simulink model "crs_controller"  (R2026b)
settings: Solver=FixedStepDiscrete  FixedStep=Ts
undefined symbols (not defined in the file): brake_threshold, DiscIntNeverNeededParam, KeyON, Kp, opMode, reqMode, ShiftDrive, target_dec_hold, target_dec_short, target_inc_hold, target_inc_short, throt_max, throt_min, Ts, tsp_max, tsp_min
libraries: simulink x73
settings Model: DataDictionary=crs_controllerdic.sldd  Creator=The MathWorks, Inc.  LastModifiedBy=alexkim
settings DataIOCC: DSMLogging=off  ReturnWorkspaceOutputs=off  SaveOutput=off  SaveTime=off  SignalLogging=off
settings OptimizationCC: DefaultParameterBehavior=Inlined  EfficientTunableParamExpr=on  PassReuseOutputArgsAs=Individual arguments
settings DebuggingCC: ArithmeticOperatorsInVariantConditions=warning  ParameterTunabilityLossMsg=error
settings SFSimCC: CustomCodeUndefinedFunction=UseInterfaceOnly  SimUseLocalCustomCode=off
settings RTWCC: DLArmComputeVersion=19.05  Description=Embedded Coder  GenCodeOnly=on  GenerateReport=on  GenerateTraceInfo=on  GenerateTraceReport=on  GenerateTraceReportEml=on  GenerateTraceReportSf=on  GenerateTraceReportSl=on  IncludeHyperlinkInReport=on  LaunchReport=on  RTWUseLocalCustomCode=off  SystemTargetFile=ert.tlc  TemplateMakefile=ert_default_tmf
settings CodeAppCC: ForceParamTrailComments=on  IgnoreCustomStorageClasses=off  InsertBlockDesc=on  MATLABFcnDesc=on  MATLABSourceComments=on  OperatorAnnotations=on  ReqsInCode=on  SFDataObjDesc=on  SimulinkDataObjDesc=on  StateflowObjectComments=on
settings ERTTargetCC: DynamicArrayContainerType=coder::array  GenerateSampleERTMain=on

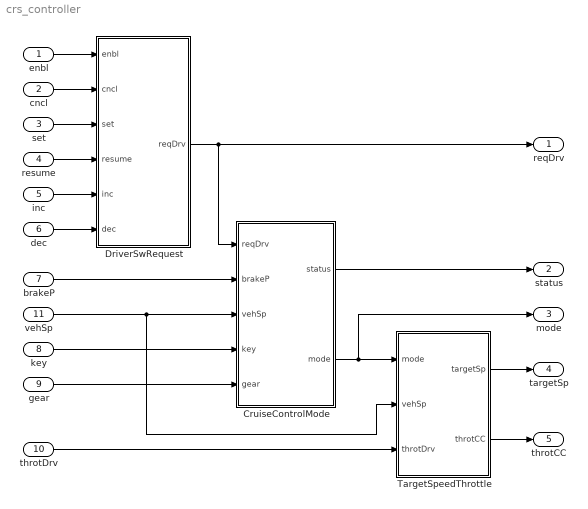
== system crs_controller ==
  enbl : Inport  OutDataTypeStr=boolean
  cncl : Inport  Port=2  OutDataTypeStr=boolean
  set : Inport  Port=3  OutDataTypeStr=boolean
  resume : Inport  Port=4  OutDataTypeStr=boolean
  inc : Inport  Port=5  OutDataTypeStr=boolean
  dec : Inport  Port=6  OutDataTypeStr=boolean
  brakeP : Inport  Port=7
  key : Inport  Port=8
  gear : Inport  Port=9  Interpolate=off
  throtDrv : Inport  Port=10
  vehSp : Inport  Port=11
  CruiseControlMode : Subsystem  RequirementInfo="{}  %GIDa_bb6d1dc8_bb76_4df1_9873_999afa682800"  TreatAsAtomicUnit=on
  DriverSwRequest : Subsystem  RequirementInfo="{}  %GIDa_29e5572c_7fa7_4cd7_a964_a3217c292b35"  TreatAsAtomicUnit=on
  TargetSpeedThrottle : Subsystem  RequirementInfo="{}  %GIDa_aedc9787_ada3_4e37_9146_515463f4d0c7"  TreatAsAtomicUnit=on
  reqDrv : Outport  VectorParamsAs1DForOutWhenUnconnected=off
  status : Outport  Port=2  VectorParamsAs1DForOutWhenUnconnected=off
  mode : Outport  Port=3  VectorParamsAs1DForOutWhenUnconnected=off
  targetSp : Outport  Port=4  VectorParamsAs1DForOutWhenUnconnected=off
  throtCC : Outport  Port=5  VectorParamsAs1DForOutWhenUnconnected=off
  wires:
  dec/1 -> DriverSwRequest/6(dec)
  inc/1 -> DriverSwRequest/5(inc)
  enbl/1 -> DriverSwRequest/1(enbl)
  vehSp/1 -> TargetSpeedThrottle/2(vehSp), CruiseControlMode/3(vehSp)
  CruiseControlMode/2(mode) -> mode/1, TargetSpeedThrottle/1(mode)
  throtDrv/1 -> TargetSpeedThrottle/3(throtDrv)
  TargetSpeedThrottle/2(throtCC) -> throtCC/1
  DriverSwRequest/1(reqDrv) -> reqDrv/1, CruiseControlMode/1(reqDrv)
  resume/1 -> DriverSwRequest/4(resume)
  set/1 -> DriverSwRequest/3(set)
  CruiseControlMode/1(status) -> status/1
  TargetSpeedThrottle/1(targetSp) -> targetSp/1
  gear/1 -> CruiseControlMode/5(gear)
  cncl/1 -> DriverSwRequest/2(cncl)
  brakeP/1 -> CruiseControlMode/2(brakeP)
  key/1 -> CruiseControlMode/4(key)

== system crs_controller/CruiseControlMode ==
  reqDrv : Inport
  brakeP : Inport  Port=2
  vehSp : Inport  Port=3
  key : Inport  Port=4
  gear : Inport  Port=5
  EnumConst2 : simulink/Sources/Enumerated Constant  OutDataTypeStr=Enum: opMode  Value=opMode.Disable  SampleTime=inf
  Switch : Switch  Criteria=u2 ~= 0  SaturateOnIntegerOverflow=off  InputSameDT=off
  UnitDelay : UnitDelay  InitialCondition=opMode.Disable  SampleTime=-1
      settings: AttributesFormatString=Init = %<InitialCondition>
  disableCaseDetection : Subsystem
  getActStatus : Subsystem
  opMode : Subsystem  TreatAsAtomicUnit=on
  outOfRange : Subsystem
  status : Outport  VectorParamsAs1DForOutWhenUnconnected=off
  mode : Outport  Port=2  VectorParamsAs1DForOutWhenUnconnected=off
  wires:
  EnumConst2/1 -> Switch/1
  brakeP/1 -> disableCaseDetection/3(brakeP)
  key/1 -> disableCaseDetection/1(key)
  gear/1 -> disableCaseDetection/2(gear)
  disableCaseDetection/1(disable_flag) -> Switch/2
  reqDrv/1 -> opMode/1(reqDrv)
  UnitDelay/1 -> opMode/3(mode_prev)  "mode_prev"
  getActStatus/1(cc_act_status) -> status/1
  opMode/1(mode) -> Switch/3  "act_mode"
  Switch/1 -> mode/1, getActStatus/1(mode), UnitDelay/1  "mode"
  vehSp/1 -> outOfRange/1(vehSp)
  outOfRange/1(outRange) -> opMode/2(outRange)

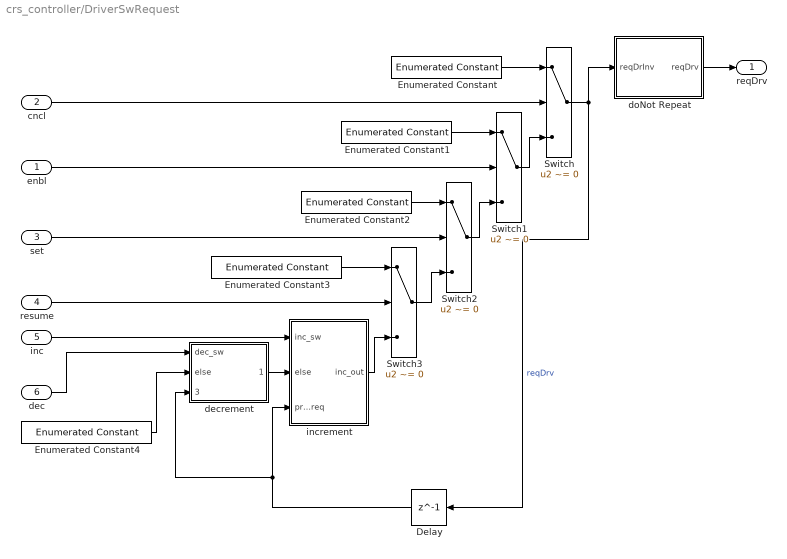
== system crs_controller/DriverSwRequest ==
  enbl : Inport
  cncl : Inport  Port=2
  set : Inport  Port=3
  resume : Inport  Port=4
  inc : Inport  Port=5  OutDataTypeStr=boolean
  dec : Inport  Port=6  OutDataTypeStr=boolean
  Delay : Delay  DelayLength=1  InitialCondition=reqMode.NoRequest
      settings: AttributesFormatString=IC: %<InitialCondition>
  Enumerated Constant : simulink/Sources/Enumerated Constant  OutDataTypeStr=Enum: reqMode  Value=reqMode.Cancel  SampleTime=inf
  Enumerated Constant1 : simulink/Sources/Enumerated Constant  OutDataTypeStr=Enum: reqMode  Value=reqMode.Cruise  SampleTime=inf
  Enumerated Constant2 : simulink/Sources/Enumerated Constant  OutDataTypeStr=Enum: reqMode  Value=reqMode.Set  SampleTime=inf
  Enumerated Constant3 : simulink/Sources/Enumerated Constant  OutDataTypeStr=Enum: reqMode  Value=reqMode.ResumeReq  SampleTime=inf
  Enumerated Constant4 : simulink/Sources/Enumerated Constant  OutDataTypeStr=Enum: reqMode  Value=reqMode.NoRequest  SampleTime=inf
  Switch : Switch  RequirementInfo="{}  %GIDa_5d0d916b_47a2_4532_93c1_fba9212dd833"  Criteria=u2 ~= 0  SaturateOnIntegerOverflow=off  InputSameDT=off
  Switch1 : Switch  RequirementInfo="{}  %GIDa_9aa713f9_64ac_4216_9525_3a0940fa8516"  Criteria=u2 ~= 0  SaturateOnIntegerOverflow=off  InputSameDT=off
  Switch2 : Switch  Criteria=u2 ~= 0  SaturateOnIntegerOverflow=off  InputSameDT=off
  Switch3 : Switch  Criteria=u2 ~= 0  SaturateOnIntegerOverflow=off  InputSameDT=off
  decrement : Subsystem
  doNot Repeat : Subsystem
  increment : Subsystem
  reqDrv : Outport  VectorParamsAs1DForOutWhenUnconnected=off
  wires:
  Enumerated Constant/1 -> Switch/1
  Switch/1 -> doNot Repeat/1(reqDrInv), Delay/1  "reqDrv"
  cncl/1 -> Switch/2
  enbl/1 -> Switch1/2
  Enumerated Constant1/1 -> Switch1/1
  Switch1/1 -> Switch/3
  set/1 -> Switch2/2
  Enumerated Constant2/1 -> Switch2/1
  resume/1 -> Switch3/2
  Enumerated Constant3/1 -> Switch3/1
  Switch3/1 -> Switch2/3
  Switch2/1 -> Switch1/3
  dec/1 -> decrement/1(dec_sw)
  Enumerated Constant4/1 -> decrement/2(else)
  inc/1 -> increment/1(inc_sw)
  decrement/1(dec_out) -> increment/2(else)
  increment/1(inc_out) -> Switch3/3
  Delay/1 -> increment/3(prev_req), decrement/3(prev_req)
  doNot Repeat/1(reqDrv) -> reqDrv/1

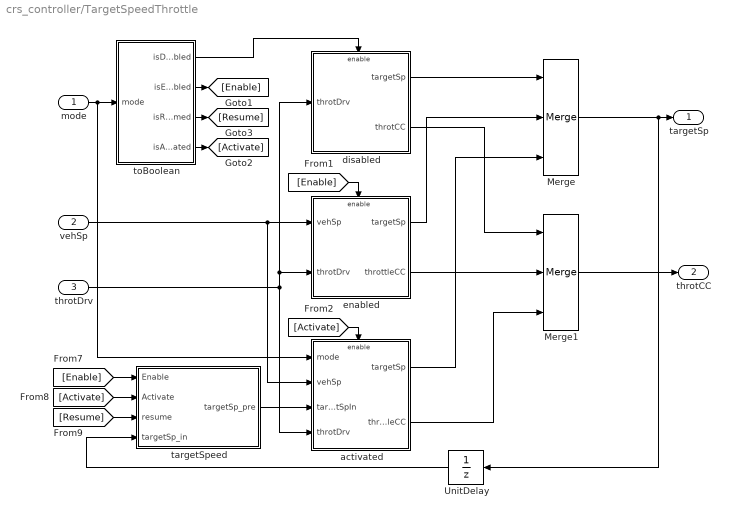
== system crs_controller/TargetSpeedThrottle ==
  mode : Inport
  vehSp : Inport  Port=2
  throtDrv : Inport  Port=3
  Merge : Merge  Inputs=3
  Merge1 : Merge  Inputs=3
  UnitDelay : UnitDelay  SampleTime=-1
      settings: AttributesFormatString=Init = %<InitialCondition>
  activated : Subsystem  TreatAsAtomicUnit=on
  disabled : Subsystem  TreatAsAtomicUnit=on
  enabled : Subsystem  TreatAsAtomicUnit=on
  targetSpeed : Subsystem
  toBoolean : Subsystem
  targetSp : Outport  VectorParamsAs1DForOutWhenUnconnected=off
  throtCC : Outport  Port=2  VectorParamsAs1DForOutWhenUnconnected=off
  wires:
  [Activate] -> targetSpeed/2(Activate)
  [Enable] -> targetSpeed/1(Enable)
  targetSpeed/1(targetSp_pre) -> activated/3(targetSpIn)
  mode/1 -> toBoolean/1(mode), activated/1(mode)
  [Activate] -> activated/Enable
  [Enable] -> enabled/Enable
  toBoolean/1(isDisabled) -> disabled/Enable
  UnitDelay/1 -> targetSpeed/4(targetSp_in)
  Merge/1 -> targetSp/1, UnitDelay/1
  throtDrv/1 -> disabled/1(throtDrv), enabled/2(throtDrv), activated/4(throtDrv)
  vehSp/1 -> activated/2(vehSp), enabled/1(vehSp)
  toBoolean/2(isEnabled) -> [Enable]
  toBoolean/3(isResumed) -> [Resume]
  toBoolean/4(isActivated) -> [Activate]
  [Resume] -> targetSpeed/3(resume)
  disabled/1(targetSp) -> Merge/1
  enabled/1(targetSp) -> Merge/2
  activated/1(targetSp) -> Merge/3
  activated/2(throttleCC) -> Merge1/3
  enabled/2(throttleCC) -> Merge1/2
  disabled/2(throtCC) -> Merge1/1
  Merge1/1 -> throtCC/1

== system crs_controller/CruiseControlMode/disableCaseDetection ==
  key : Inport
  gear : Inport  Port=2
  brakeP : Inport  Port=3
  IsKeyPositionOn : Subsystem
  IsShiftDrive : Subsystem
  LogicOp1 : Logic  Operator=OR  Inputs=3  AllPortsSameDT=off  OutDataTypeStr=boolean
  isbrake : Subsystem
  disable_flag : Outport  VectorParamsAs1DForOutWhenUnconnected=off
  wires:
  LogicOp1/1 -> disable_flag/1
  brakeP/1 -> isbrake/1(brakeP)
  isbrake/1(isbrake) -> LogicOp1/3  "isbrake"
  key/1 -> IsKeyPositionOn/1(In1)
  IsKeyPositionOn/1(Out1) -> LogicOp1/1
  gear/1 -> IsShiftDrive/1(In1)
  IsShiftDrive/1(Out1) -> LogicOp1/2

== system crs_controller/CruiseControlMode/getActStatus ==
  mode : Inport
  EnumConst1 : simulink/Sources/Enumerated Constant  OutDataTypeStr=Enum: opMode  Value=opMode.Disable  SampleTime=inf
  EnumConst2 : simulink/Sources/Enumerated Constant  OutDataTypeStr=Enum: opMode  Value=opMode.Enable  SampleTime=inf
  LogicOp1 : Logic  AllPortsSameDT=off  OutDataTypeStr=boolean
  Relational Operator1 : RelationalOperator  Operator=~=  OutDataTypeStr=boolean  InputSameDT=off
  Relational Operator2 : RelationalOperator  Operator=~=  OutDataTypeStr=boolean  InputSameDT=off
  cc_act_status : Outport  VectorParamsAs1DForOutWhenUnconnected=off
  wires:
  Relational Operator2/1 -> LogicOp1/1
  EnumConst1/1 -> Relational Operator2/1
  mode/1 -> Relational Operator1/2, Relational Operator2/2
  Relational Operator1/1 -> LogicOp1/2
  EnumConst2/1 -> Relational Operator1/1
  LogicOp1/1 -> cc_act_status/1

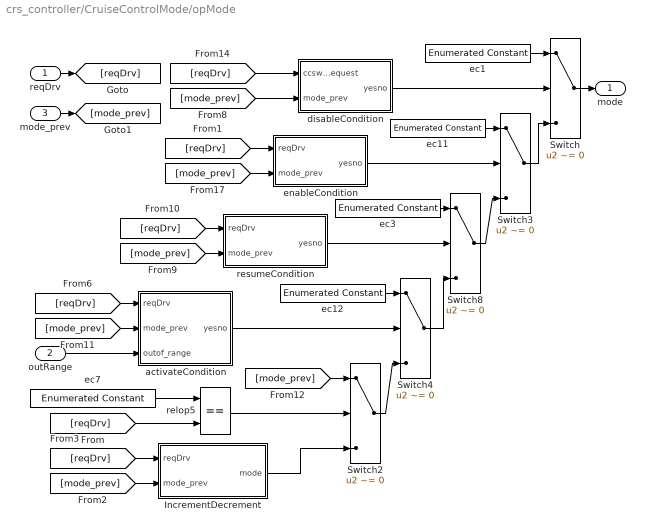
== system crs_controller/CruiseControlMode/opMode ==
  reqDrv : Inport
  outRange : Inport  Port=2
  mode_prev : Inport  Port=3
  IncrementDecrement : Subsystem
  Switch{,2..4,8} (5 alike) : Switch  Criteria=u2 ~= 0  SaturateOnIntegerOverflow=off  InputSameDT=off
  activateCondition : Subsystem
  disableCondition : Subsystem
  ec1 : simulink/Sources/Enumerated Constant  OutDataTypeStr=Enum: opMode  Value=opMode.Disable  SampleTime=inf
  ec11 : simulink/Sources/Enumerated Constant  OutDataTypeStr=Enum: opMode  Value=opMode.Enable  SampleTime=inf
  ec12 : simulink/Sources/Enumerated Constant  OutDataTypeStr=Enum: opMode  Value=opMode.Activate  SampleTime=inf
  ec3 : simulink/Sources/Enumerated Constant  OutDataTypeStr=Enum: opMode  Value=opMode.Resume  SampleTime=inf
  ec7 : simulink/Sources/Enumerated Constant  OutDataTypeStr=Enum: reqMode  Value=reqMode.NoRequest  SampleTime=inf
  enableCondition : Subsystem
  relop5 : RelationalOperator  Operator===  OutDataTypeStr=boolean  InputSameDT=off
  resumeCondition : Subsystem
  mode : Outport  VectorParamsAs1DForOutWhenUnconnected=off
  wires:
  Switch/1 -> mode/1
  ec1/1 -> Switch/1
  ec7/1 -> relop5/1
  ec11/1 -> Switch3/1
  ec12/1 -> Switch4/1
  [reqDrv] -> relop5/2
  [mode_prev] -> Switch2/1
  [reqDrv] -> enableCondition/1(reqDrv)
  mode_prev/1 -> [mode_prev]
  enableCondition/1(yesno) -> Switch3/2
  disableCondition/1(yesno) -> Switch/2
  Switch3/1 -> Switch/3
  activateCondition/1(yesno) -> Switch4/2
  [reqDrv] -> activateCondition/1(reqDrv)
  [mode_prev] -> activateCondition/2(mode_prev)
  [mode_prev] -> disableCondition/2(mode_prev)
  reqDrv/1 -> [reqDrv]
  relop5/1 -> Switch2/2
  Switch2/1 -> Switch4/3
  Switch8/1 -> Switch3/3
  Switch4/1 -> Switch8/3
  resumeCondition/1(yesno) -> Switch8/2
  [mode_prev] -> resumeCondition/2(mode_prev)
  [reqDrv] -> resumeCondition/1(reqDrv)
  ec3/1 -> Switch8/1
  [reqDrv] -> disableCondition/1(ccsw_request)
  outRange/1 -> activateCondition/3(outof_range)
  [mode_prev] -> enableCondition/2(mode_prev)
  [reqDrv] -> IncrementDecrement/1(reqDrv)
  [mode_prev] -> IncrementDecrement/2(mode_prev)
  IncrementDecrement/1(mode) -> Switch2/3

== system crs_controller/CruiseControlMode/outOfRange ==
  vehSp : Inport
  Compare To Constant : simulink/Logic and Bit Operations/Compare To Constant  relop=<  const=tsp_min  OutDataTypeStr=boolean
  Compare To Constant1 : simulink/Logic and Bit Operations/Compare To Constant  relop=>  const=tsp_max  OutDataTypeStr=boolean
  LogicOp : Logic  Operator=OR  AllPortsSameDT=off  OutDataTypeStr=boolean
  outRange : Outport  VectorParamsAs1DForOutWhenUnconnected=off
  wires:
  LogicOp/1 -> outRange/1
  Compare To Constant1/1 -> LogicOp/2
  Compare To Constant/1 -> LogicOp/1
  vehSp/1 -> Compare To Constant/1, Compare To Constant1/1

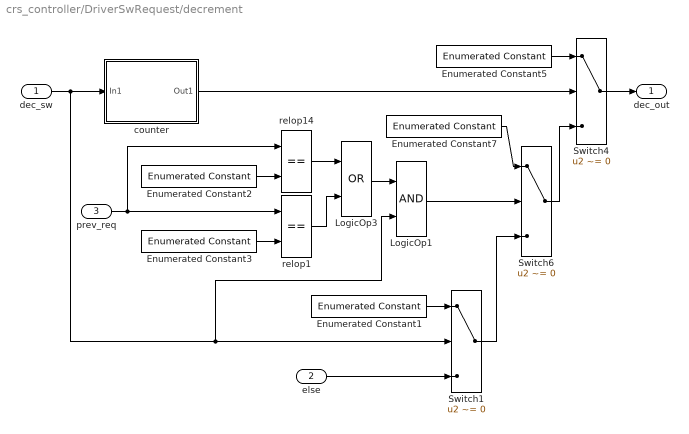
== system crs_controller/DriverSwRequest/decrement ==
  dec_sw : Inport
  else : Inport  Port=2
  prev_req : Inport  Port=3
  Enumerated Constant1 : simulink/Sources/Enumerated Constant  OutDataTypeStr=Enum: reqMode  Value=reqMode.Dec_Short  SampleTime=inf
  Enumerated Constant2 : simulink/Sources/Enumerated Constant  OutDataTypeStr=Enum: reqMode  Value=reqMode.Dec_Short  SampleTime=inf
  Enumerated Constant3 : simulink/Sources/Enumerated Constant  OutDataTypeStr=Enum: reqMode  Value=reqMode.Dec_Middle  SampleTime=inf
  Enumerated Constant5 : simulink/Sources/Enumerated Constant  OutDataTypeStr=Enum: reqMode  Value=reqMode.Dec_Long  SampleTime=inf
  Enumerated Constant7 : simulink/Sources/Enumerated Constant  OutDataTypeStr=Enum: reqMode  Value=reqMode.Dec_Middle  SampleTime=inf
  LogicOp1 : Logic  AllPortsSameDT=off  OutDataTypeStr=boolean
  LogicOp3 : Logic  Operator=OR  AllPortsSameDT=off  OutDataTypeStr=boolean
  Switch1 : Switch  Criteria=u2 ~= 0  SaturateOnIntegerOverflow=off  InputSameDT=off
  Switch4 : Switch  Criteria=u2 ~= 0  SaturateOnIntegerOverflow=off  InputSameDT=off
  Switch6 : Switch  Criteria=u2 ~= 0  SaturateOnIntegerOverflow=off  InputSameDT=off
  counter : Subsystem  DisableCoverage=on  mask(SLDV counter){CountValue=50, OutDataTypeStr=uint8}
      mask prompts: CountValue "Count value"; OutDataTypeStr "Data type"
      mask help: A counter block optimized for Simulink Design Verifier test case generation. If the input is true for consecutive steps which is specified the Count value parameter, then the output is TRUE, otherwise it is FALSE.
      mask init:
      | if CountValue < 0 || CountValue > intmax(OutDataTypeStr)
      |     error('Specified count value needs to be within 0-%d.',intmax(OutDataTypeStr))
      | end
      mask Display: disp(sprintf('Counter (%s)\nCount:%d',OutDataTypeStr,CountValue))
  relop1 : RelationalOperator  Operator===  OutDataTypeStr=boolean  InputSameDT=off
  relop14 : RelationalOperator  Operator===  OutDataTypeStr=boolean  InputSameDT=off
  dec_out : Outport  VectorParamsAs1DForOutWhenUnconnected=off
  wires:
  Enumerated Constant5/1 -> Switch4/1
  Switch4/1 -> dec_out/1
  Enumerated Constant7/1 -> Switch6/1
  Switch6/1 -> Switch4/3
  counter/1(Out1) -> Switch4/2
  Switch1/1 -> Switch6/3
  dec_sw/1 -> counter/1(In1), LogicOp1/2, Switch1/2
  else/1 -> Switch1/3
  Enumerated Constant1/1 -> Switch1/1
  Enumerated Constant2/1 -> relop14/2
  Enumerated Constant3/1 -> relop1/2
  prev_req/1 -> relop14/1, relop1/1
  relop14/1 -> LogicOp3/1
  relop1/1 -> LogicOp3/2
  LogicOp3/1 -> LogicOp1/1
  LogicOp1/1 -> Switch6/2

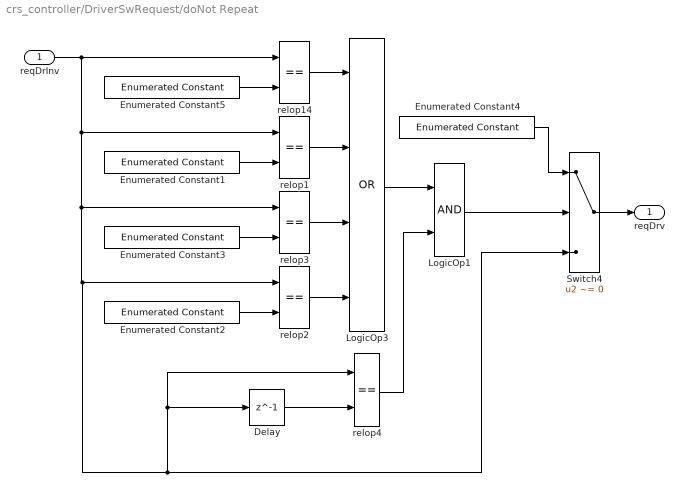
== system crs_controller/DriverSwRequest/doNot Repeat ==
  reqDrInv : Inport
  Delay : Delay  DelayLength=1  InitialCondition=reqMode.NoRequest
      settings: AttributesFormatString=Init = %<InitialCondition>
  Enumerated Constant1 : simulink/Sources/Enumerated Constant  OutDataTypeStr=Enum: reqMode  Value=reqMode.Cruise  SampleTime=inf
  Enumerated Constant2 : simulink/Sources/Enumerated Constant  OutDataTypeStr=Enum: reqMode  Value=reqMode.ResumeReq  SampleTime=inf
  Enumerated Constant3 : simulink/Sources/Enumerated Constant  OutDataTypeStr=Enum: reqMode  Value=reqMode.Set  SampleTime=inf
  Enumerated Constant4 : simulink/Sources/Enumerated Constant  OutDataTypeStr=Enum: reqMode  Value=reqMode.NoRequest  SampleTime=inf
  Enumerated Constant5 : simulink/Sources/Enumerated Constant  OutDataTypeStr=Enum: reqMode  Value=reqMode.Cancel  SampleTime=inf
  LogicOp1 : Logic  AllPortsSameDT=off  OutDataTypeStr=boolean
  LogicOp3 : Logic  Operator=OR  Inputs=4  AllPortsSameDT=off  OutDataTypeStr=boolean
  Switch4 : Switch  Criteria=u2 ~= 0  SaturateOnIntegerOverflow=off  InputSameDT=off
  relop{1..4,14} (5 alike) : RelationalOperator  Operator===  OutDataTypeStr=boolean  InputSameDT=off
  reqDrv : Outport  VectorParamsAs1DForOutWhenUnconnected=off
  wires:
  Enumerated Constant5/1 -> relop14/2
  Enumerated Constant1/1 -> relop1/2
  Enumerated Constant3/1 -> relop3/2
  Enumerated Constant2/1 -> relop2/2
  reqDrInv/1 -> Switch4/3, relop4/1, Delay/1, relop2/1, relop3/1, relop1/1, relop14/1
  relop14/1 -> LogicOp3/1
  relop1/1 -> LogicOp3/2
  relop3/1 -> LogicOp3/3
  relop2/1 -> LogicOp3/4
  Switch4/1 -> reqDrv/1
  Delay/1 -> relop4/2
  relop4/1 -> LogicOp1/2
  LogicOp3/1 -> LogicOp1/1
  LogicOp1/1 -> Switch4/2
  Enumerated Constant4/1 -> Switch4/1

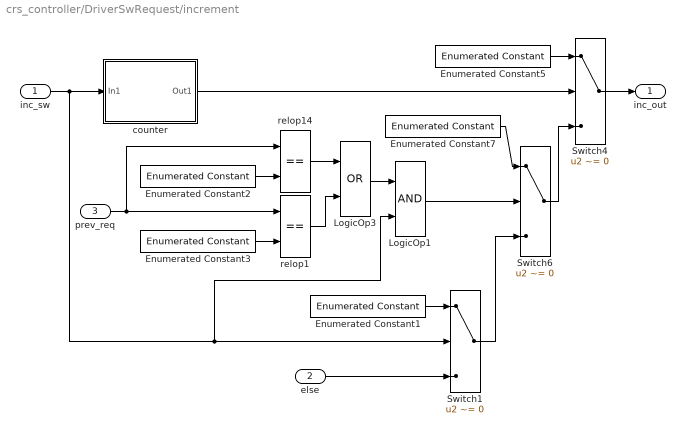
== system crs_controller/DriverSwRequest/increment ==
  inc_sw : Inport
  else : Inport  Port=2
  prev_req : Inport  Port=3
  Enumerated Constant1 : simulink/Sources/Enumerated Constant  OutDataTypeStr=Enum: reqMode  Value=reqMode.Inc_Short  SampleTime=inf
  Enumerated Constant2 : simulink/Sources/Enumerated Constant  OutDataTypeStr=Enum: reqMode  Value=reqMode.Inc_Short  SampleTime=inf
  Enumerated Constant3 : simulink/Sources/Enumerated Constant  OutDataTypeStr=Enum: reqMode  Value=reqMode.Inc_Middle  SampleTime=inf
  Enumerated Constant5 : simulink/Sources/Enumerated Constant  OutDataTypeStr=Enum: reqMode  Value=reqMode.Inc_Long  SampleTime=inf
  Enumerated Constant7 : simulink/Sources/Enumerated Constant  OutDataTypeStr=Enum: reqMode  Value=reqMode.Inc_Middle  SampleTime=inf
  LogicOp1 : Logic  AllPortsSameDT=off  OutDataTypeStr=boolean
  LogicOp3 : Logic  Operator=OR  AllPortsSameDT=off  OutDataTypeStr=boolean
  Switch1 : Switch  Criteria=u2 ~= 0  SaturateOnIntegerOverflow=off  InputSameDT=off
  Switch4 : Switch  Criteria=u2 ~= 0  SaturateOnIntegerOverflow=off  InputSameDT=off
  Switch6 : Switch  Criteria=u2 ~= 0  SaturateOnIntegerOverflow=off  InputSameDT=off
  counter : Subsystem  DisableCoverage=on  mask(SLDV counter){CountValue=50, OutDataTypeStr=uint8}
      mask prompts: CountValue "Count value"; OutDataTypeStr "Data type"
      mask help: A counter block optimized for Simulink Design Verifier test case generation. If the input is true for consecutive steps which is specified the Count value parameter, then the output is TRUE, otherwise it is FALSE.
      mask init:
      | if CountValue < 0 || CountValue > intmax(OutDataTypeStr)
      |     error('Specified count value needs to be within 0-%d.',intmax(OutDataTypeStr))
      | end
      mask Display: disp(sprintf('Counter (%s)\nCount:%d',OutDataTypeStr,CountValue))
  relop1 : RelationalOperator  Operator===  OutDataTypeStr=boolean  InputSameDT=off
  relop14 : RelationalOperator  Operator===  OutDataTypeStr=boolean  InputSameDT=off
  inc_out : Outport  VectorParamsAs1DForOutWhenUnconnected=off
  wires:
  Enumerated Constant5/1 -> Switch4/1
  Switch4/1 -> inc_out/1
  Enumerated Constant7/1 -> Switch6/1
  Switch6/1 -> Switch4/3
  counter/1(Out1) -> Switch4/2
  Switch1/1 -> Switch6/3
  inc_sw/1 -> counter/1(In1), LogicOp1/2, Switch1/2
  else/1 -> Switch1/3
  Enumerated Constant1/1 -> Switch1/1
  Enumerated Constant2/1 -> relop14/2
  Enumerated Constant3/1 -> relop1/2
  prev_req/1 -> relop14/1, relop1/1
  relop14/1 -> LogicOp3/1
  relop1/1 -> LogicOp3/2
  LogicOp3/1 -> LogicOp1/1
  LogicOp1/1 -> Switch6/2

== system crs_controller/TargetSpeedThrottle/activated ==
  mode : Inport
  vehSp : Inport  Port=2
  targetSpIn : Inport  Port=3
  throtDrv : Inport  Port=4
  Enable : EnablePort
  getNewTargetSpeed : Subsystem
  getThrottleValue : Subsystem
  targetSp : Outport  VectorParamsAs1DForOutWhenUnconnected=off
  throttleCC : Outport  Port=2  VectorParamsAs1DForOutWhenUnconnected=off
  wires:
  targetSpIn/1 -> getThrottleValue/1(In1), getNewTargetSpeed/1(targetSpIn)
  mode/1 -> getNewTargetSpeed/2(mode)
  getNewTargetSpeed/1(targetSp) -> targetSp/1  "targetSp"
  vehSp/1 -> getThrottleValue/2(In2)
  throtDrv/1 -> getThrottleValue/3(In3)
  getThrottleValue/1(Out1) -> throttleCC/1

== system crs_controller/TargetSpeedThrottle/disabled ==
  throtDrv : Inport
  Enable : EnablePort
  Constant : Constant  Value=tsp_min  OutDataTypeStr=Inherit: Inherit via back propagation
  targetSp : Outport  VectorParamsAs1DForOutWhenUnconnected=off
  throtCC : Outport  Port=2  VectorParamsAs1DForOutWhenUnconnected=off
  wires:
  Constant/1 -> targetSp/1
  throtDrv/1 -> throtCC/1

== system crs_controller/TargetSpeedThrottle/enabled ==
  vehSp : Inport
  throtDrv : Inport  Port=2
  Enable : EnablePort
  targetSp : Outport  VectorParamsAs1DForOutWhenUnconnected=off
  throttleCC : Outport  Port=2  VectorParamsAs1DForOutWhenUnconnected=off
  wires:
  vehSp/1 -> targetSp/1
  throtDrv/1 -> throttleCC/1

== system crs_controller/TargetSpeedThrottle/targetSpeed ==
  Enable : Inport
  Activate : Inport  Port=2
  resume : Inport  Port=3
  targetSp_in : Inport  Port=4
  LogicOp1 : Logic  AllPortsSameDT=off  OutDataTypeStr=boolean
  Switch5 : Switch  Criteria=u2 ~= 0  SaturateOnIntegerOverflow=off  InputSameDT=off
  UnitDelay1 : UnitDelay  InitialCondition=false  SampleTime=-1
      settings: AttributesFormatString=Init = %<InitialCondition>
  storeSpeed : Subsystem  TreatAsAtomicUnit=on
  targetSp_pre : Outport  VectorParamsAs1DForOutWhenUnconnected=off
  wires:
  storeSpeed/1(stored_targetSp) -> Switch5/1
  Activate/1 -> UnitDelay1/1
  UnitDelay1/1 -> LogicOp1/2
  LogicOp1/1 -> storeSpeed/Enable
  Enable/1 -> LogicOp1/1
  resume/1 -> Switch5/2
  targetSp_in/1 -> Switch5/3, storeSpeed/1(targetSp_prev)
  Switch5/1 -> targetSp_pre/1

== system crs_controller/TargetSpeedThrottle/toBoolean ==
  mode : Inport
  EnumConst1 : simulink/Sources/Enumerated Constant  OutDataTypeStr=Enum: opMode  Value=opMode.Disable  SampleTime=inf
  EnumConst2 : simulink/Sources/Enumerated Constant  OutDataTypeStr=Enum: opMode  Value=opMode.Resume  SampleTime=inf
  EnumConst3 : simulink/Sources/Enumerated Constant  OutDataTypeStr=Enum: opMode  Value=opMode.Enable  SampleTime=inf
  LogicOp : Logic  Operator=NOR  Inputs=3  AllPortsSameDT=off  OutDataTypeStr=boolean
  relop1 : RelationalOperator  Operator===  OutDataTypeStr=boolean  InputSameDT=off
  relop2 : RelationalOperator  Operator===  OutDataTypeStr=boolean  InputSameDT=off
  relop3 : RelationalOperator  Operator===  OutDataTypeStr=boolean  InputSameDT=off
  isDisabled : Outport  VectorParamsAs1DForOutWhenUnconnected=off
  isEnabled : Outport  Port=2  VectorParamsAs1DForOutWhenUnconnected=off
  isResumed : Outport  Port=3  VectorParamsAs1DForOutWhenUnconnected=off
  isActivated : Outport  Port=4  VectorParamsAs1DForOutWhenUnconnected=off
  wires:
  relop3/1 -> isResumed/1, LogicOp/3
  EnumConst2/1 -> relop3/1
  LogicOp/1 -> isActivated/1
  relop2/1 -> isEnabled/1, LogicOp/2
  EnumConst3/1 -> relop2/1
  relop1/1 -> isDisabled/1, LogicOp/1
  EnumConst1/1 -> relop1/1
  mode/1 -> relop2/2, relop3/2, relop1/2

== system crs_controller/CruiseControlMode/disableCaseDetection/IsKeyPositionOn ==
  In1 : Inport
  Constant : Constant  Value=KeyON
  Relational Operator2 : RelationalOperator  Operator=~=  OutDataTypeStr=boolean  InputSameDT=off
  Out1 : Outport  VectorParamsAs1DForOutWhenUnconnected=off
  wires:
  Relational Operator2/1 -> Out1/1
  In1/1 -> Relational Operator2/1
  Constant/1 -> Relational Operator2/2

== system crs_controller/CruiseControlMode/disableCaseDetection/IsShiftDrive ==
  In1 : Inport
  Constant1 : Constant  Value=ShiftDrive
  Relational Operator3 : RelationalOperator  Operator=~=  OutDataTypeStr=boolean  InputSameDT=off
  Out1 : Outport  VectorParamsAs1DForOutWhenUnconnected=off
  wires:
  Relational Operator3/1 -> Out1/1
  In1/1 -> Relational Operator3/1
  Constant1/1 -> Relational Operator3/2

== system crs_controller/CruiseControlMode/disableCaseDetection/isbrake ==
  brakeP : Inport
  Compare To Constant : simulink/Logic and Bit Operations/Compare To Constant  relop=>  const=brake_threshold  OutDataTypeStr=boolean
  isbrake : Outport  VectorParamsAs1DForOutWhenUnconnected=off
  wires:
  brakeP/1 -> Compare To Constant/1
  Compare To Constant/1 -> isbrake/1

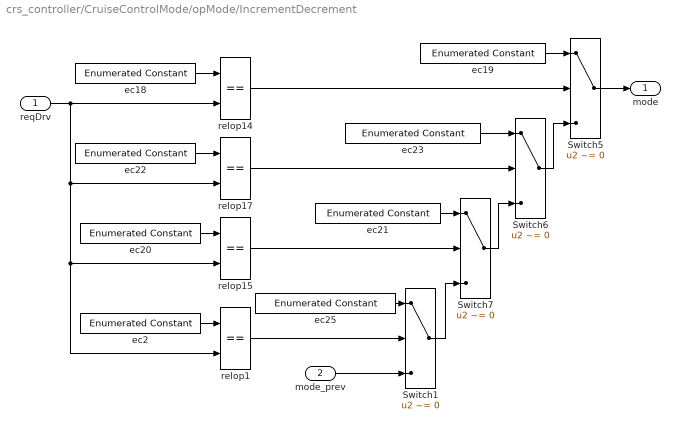
== system crs_controller/CruiseControlMode/opMode/IncrementDecrement ==
  reqDrv : Inport
  mode_prev : Inport  Port=2
  Switch{1,5..7} (4 alike) : Switch  Criteria=u2 ~= 0  SaturateOnIntegerOverflow=off  InputSameDT=off
  ec18 : simulink/Sources/Enumerated Constant  OutDataTypeStr=Enum: reqMode  Value=reqMode.Inc_Short  SampleTime=inf
  ec19 : simulink/Sources/Enumerated Constant  OutDataTypeStr=Enum: opMode  Value=opMode.Increment  SampleTime=inf
  ec2 : simulink/Sources/Enumerated Constant  OutDataTypeStr=Enum: reqMode  Value=reqMode.Dec_Long  SampleTime=inf
  ec20 : simulink/Sources/Enumerated Constant  OutDataTypeStr=Enum: reqMode  Value=reqMode.Dec_Short  SampleTime=inf
  ec21 : simulink/Sources/Enumerated Constant  OutDataTypeStr=Enum: opMode  Value=opMode.Decrement  SampleTime=inf
  ec22 : simulink/Sources/Enumerated Constant  OutDataTypeStr=Enum: reqMode  Value=reqMode.Inc_Long  SampleTime=inf
  ec23 : simulink/Sources/Enumerated Constant  OutDataTypeStr=Enum: opMode  Value=opMode.IncrementHold  SampleTime=inf
  ec25 : simulink/Sources/Enumerated Constant  OutDataTypeStr=Enum: opMode  Value=opMode.DecrementHold  SampleTime=inf
  relop{1,14..15,17} (4 alike) : RelationalOperator  Operator===  OutDataTypeStr=boolean  InputSameDT=off
  mode : Outport  VectorParamsAs1DForOutWhenUnconnected=off
  wires:
  ec19/1 -> Switch5/1
  ec22/1 -> relop17/1
  relop17/1 -> Switch6/2
  ec23/1 -> Switch6/1
  Switch6/1 -> Switch5/3
  ec20/1 -> relop15/1
  relop15/1 -> Switch7/2
  ec21/1 -> Switch7/1
  Switch7/1 -> Switch6/3
  ec25/1 -> Switch1/1
  Switch1/1 -> Switch7/3
  ec2/1 -> relop1/1
  relop1/1 -> Switch1/2
  mode_prev/1 -> Switch1/3
  ec18/1 -> relop14/1
  relop14/1 -> Switch5/2
  Switch5/1 -> mode/1
  reqDrv/1 -> relop1/2, relop15/2, relop17/2, relop14/2

== system crs_controller/CruiseControlMode/opMode/activateCondition ==
  reqDrv : Inport
  mode_prev : Inport  Port=2
  outof_range : Inport  Port=3
  LogicOp5 : Logic  Operator=OR  Inputs=4  AllPortsSameDT=off  OutDataTypeStr=boolean
  activate : Subsystem
  keepActivated : Subsystem
  resumeToActive : Subsystem
  waitingForButtonHolding : Subsystem
  yesno : Outport  VectorParamsAs1DForOutWhenUnconnected=off
  wires:
  reqDrv/1 -> keepActivated/1(reqDrv), waitingForButtonHolding/1(reqDrv), activate/1(reqDrv)
  LogicOp5/1 -> yesno/1
  outof_range/1 -> activate/2(outof_range)
  keepActivated/1(yesno) -> LogicOp5/3
  waitingForButtonHolding/1(yesno) -> LogicOp5/2  "toBeHoldState"
  activate/1(yesno) -> LogicOp5/1  "toBeActivated"
  resumeToActive/1(yesno) -> LogicOp5/4
  mode_prev/1 -> keepActivated/2(mode_prev), resumeToActive/1(mode_prev)

== system crs_controller/CruiseControlMode/opMode/disableCondition ==
  ccsw_request : Inport
  mode_prev : Inport  Port=2
  LogicOp7 : Logic  Operator=OR  AllPortsSameDT=off  OutDataTypeStr=boolean
  buttonsShouldBeCalledWhenActivated : Subsystem
  turnOffCruise : Subsystem
  yesno : Outport  VectorParamsAs1DForOutWhenUnconnected=off
  wires:
  ccsw_request/1 -> buttonsShouldBeCalledWhenActivated/1(ccsw_request), turnOffCruise/1(ccsw_request)
  LogicOp7/1 -> yesno/1
  mode_prev/1 -> buttonsShouldBeCalledWhenActivated/2(mode_prev), turnOffCruise/2(mode_prev)
  turnOffCruise/1(yesno) -> LogicOp7/1
  buttonsShouldBeCalledWhenActivated/1(yesno) -> LogicOp7/2

== system crs_controller/CruiseControlMode/opMode/enableCondition ==
  reqDrv : Inport
  mode_prev : Inport  Port=2
  LogicOp4 : Logic  Operator=OR  AllPortsSameDT=off  OutDataTypeStr=boolean
  cancelActivation : Subsystem
  pressSetSw : Subsystem
  yesno : Outport  VectorParamsAs1DForOutWhenUnconnected=off
  wires:
  LogicOp4/1 -> yesno/1
  reqDrv/1 -> cancelActivation/1(reqDrv), pressSetSw/1(reqDrv)
  cancelActivation/1(yesno) -> LogicOp4/2
  mode_prev/1 -> cancelActivation/2(mode_prev)
  pressSetSw/1(yesno) -> LogicOp4/1

== system crs_controller/CruiseControlMode/opMode/resumeCondition ==
  reqDrv : Inport
  mode_prev : Inport  Port=2
  LogicOp6 : Logic  AllPortsSameDT=off  OutDataTypeStr=boolean
  enableToResume : Subsystem
  hasCanceled : Subsystem
  yesno : Outport  VectorParamsAs1DForOutWhenUnconnected=off
  wires:
  LogicOp6/1 -> yesno/1
  mode_prev/1 -> enableToResume/2(mode_prev), hasCanceled/1(mode_prev)
  hasCanceled/1(yesno) -> LogicOp6/2
  enableToResume/1(yesno) -> LogicOp6/1
  reqDrv/1 -> enableToResume/1(reqDrv)

== system crs_controller/DriverSwRequest/decrement/counter ==
  In1 : Inport
  Constant : Constant  Value=CountValue  OutDataTypeStr=OutDataTypeStr
  counter : MATLAB Function  TreatAsAtomicUnit=on
  Out1 : Outport  VectorParamsAs1DForOutWhenUnconnected=off
  wires:
  Constant/1 -> counter/2(CountValue)
  counter/1(out) -> Out1/1
  In1/1 -> counter/1(in)

== system crs_controller/DriverSwRequest/increment/counter ==
  In1 : Inport
  Constant : Constant  Value=CountValue  OutDataTypeStr=OutDataTypeStr
  counter : MATLAB Function  TreatAsAtomicUnit=on
  Out1 : Outport  VectorParamsAs1DForOutWhenUnconnected=off
  wires:
  Constant/1 -> counter/2(CountValue)
  counter/1(out) -> Out1/1
  In1/1 -> counter/1(in)

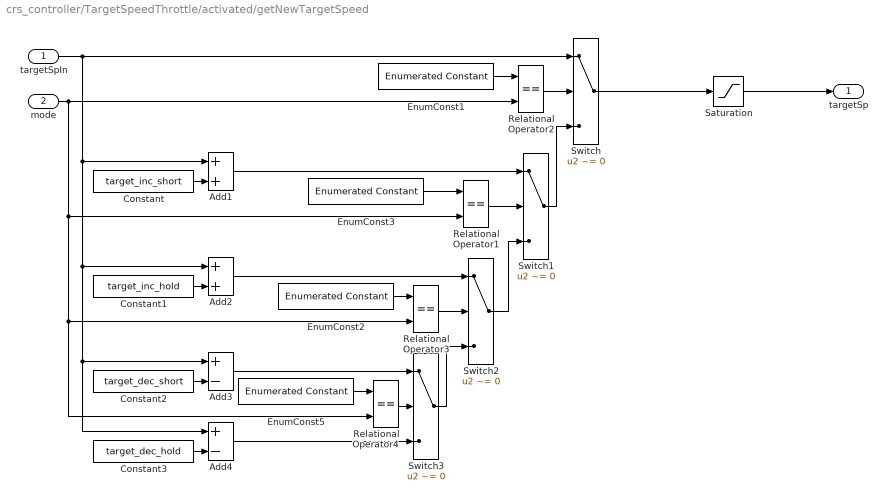
== system crs_controller/TargetSpeedThrottle/activated/getNewTargetSpeed ==
  targetSpIn : Inport
  mode : Inport  Port=2
  Add1 : Sum
  Add2 : Sum
  Add3 : Sum  Inputs=+-
  Add4 : Sum  Inputs=+-
  Constant : Constant  Value=target_inc_short  OutDataTypeStr=Inherit: Inherit via back propagation
  Constant1 : Constant  Value=target_inc_hold  OutDataTypeStr=Inherit: Inherit via back propagation
  Constant2 : Constant  Value=target_dec_short  OutDataTypeStr=Inherit: Inherit via back propagation
  Constant3 : Constant  Value=target_dec_hold  OutDataTypeStr=Inherit: Inherit via back propagation
  EnumConst1 : simulink/Sources/Enumerated Constant  OutDataTypeStr=Enum: opMode  Value=opMode.Activate  SampleTime=inf
  EnumConst2 : simulink/Sources/Enumerated Constant  OutDataTypeStr=Enum: opMode  Value=opMode.IncrementHold  SampleTime=inf
  EnumConst3 : simulink/Sources/Enumerated Constant  OutDataTypeStr=Enum: opMode  Value=opMode.Increment  SampleTime=inf
  EnumConst5 : simulink/Sources/Enumerated Constant  OutDataTypeStr=Enum: opMode  Value=opMode.Decrement  SampleTime=inf
  Relational Operator{1..4} (4 alike) : RelationalOperator  Operator===  OutDataTypeStr=boolean  InputSameDT=off
  Saturation : Saturate  UpperLimit=tsp_max  LowerLimit=tsp_min
      settings: AttributesFormatString=|
      | H:%<UpperLimit>
      | L:%<LowerLimit>
  Switch{,1..3} (4 alike) : Switch  Criteria=u2 ~= 0  SaturateOnIntegerOverflow=off  InputSameDT=off
  targetSp : Outport  VectorParamsAs1DForOutWhenUnconnected=off
  wires:
  targetSpIn/1 -> Switch/1, Add1/1, Add4/1, Add3/1, Add2/1
  Switch3/1 -> Switch2/3
  Add4/1 -> Switch3/3
  EnumConst2/1 -> Relational Operator3/1
  mode/1 -> Relational Operator4/2, Relational Operator3/2, Relational Operator1/2, Relational Operator2/2
  EnumConst1/1 -> Relational Operator2/1
  EnumConst3/1 -> Relational Operator1/1
  Constant3/1 -> Add4/2
  Constant2/1 -> Add3/2
  EnumConst5/1 -> Relational Operator4/1
  Relational Operator4/1 -> Switch3/2
  Add3/1 -> Switch3/1
  Constant1/1 -> Add2/2
  Add2/1 -> Switch2/1
  Add1/1 -> Switch1/1
  Relational Operator3/1 -> Switch2/2
  Constant/1 -> Add1/2
  Switch2/1 -> Switch1/3
  Switch1/1 -> Switch/3
  Relational Operator1/1 -> Switch1/2
  Switch/1 -> Saturation/1
  Relational Operator2/1 -> Switch/2
  Saturation/1 -> targetSp/1

== system crs_controller/TargetSpeedThrottle/activated/getThrottleValue ==
  In1 : Inport
  In2 : Inport  Port=2
  In3 : Inport  Port=3
  Delay1 : Delay  DelayLength=1  InitialCondition=0
      settings: AttributesFormatString=Init = %<InitialCondition>
  PI controller : Subsystem  TreatAsAtomicUnit=on
  Saturation2 : Saturate  UpperLimit=throt_max  LowerLimit=throt_min
      settings: AttributesFormatString=|
      | H:%<UpperLimit>
      | L:%<LowerLimit>
  Switch : Switch  Criteria=u2 ~= 0  SaturateOnIntegerOverflow=off  InputSameDT=off
  UsePI : Subsystem
  Out1 : Outport  VectorParamsAs1DForOutWhenUnconnected=off
  wires:
  In3/1 -> UsePI/4(throtDrv), Switch/3
  Delay1/1 -> PI controller/Enable
  UsePI/1(yesno) -> Delay1/1, Switch/2
  In2/1 -> UsePI/3(vehSp), PI controller/2(vehSp)
  Saturation2/1 -> Out1/1
  PI controller/1(throt) -> UsePI/1(throtPI), Switch/1
  Switch/1 -> Saturation2/1
  In1/1 -> UsePI/2(targetSpIn), PI controller/1(targetSpIn)

== system crs_controller/TargetSpeedThrottle/targetSpeed/storeSpeed ==
  targetSp_prev : Inport
  Enable : EnablePort
  stored_targetSp : Outport  VectorParamsAs1DForOutWhenUnconnected=off
  wires:
  targetSp_prev/1 -> stored_targetSp/1

== system crs_controller/CruiseControlMode/opMode/activateCondition/activate ==
  reqDrv : Inport
  outof_range : Inport  Port=2
  LogicOp3 : Logic  AllPortsSameDT=off  OutDataTypeStr=boolean
  LogicOp5 : Logic  Operator=NOT  AllPortsSameDT=off  OutDataTypeStr=boolean
  ec15 : simulink/Sources/Enumerated Constant  OutDataTypeStr=Enum: reqMode  Value=reqMode.Set  SampleTime=inf
  relop11 : RelationalOperator  Operator===  OutDataTypeStr=boolean  InputSameDT=off
  yesno : Outport  VectorParamsAs1DForOutWhenUnconnected=off
  wires:
  ec15/1 -> relop11/1
  reqDrv/1 -> relop11/2
  LogicOp3/1 -> yesno/1
  relop11/1 -> LogicOp3/1
  outof_range/1 -> LogicOp5/1
  LogicOp5/1 -> LogicOp3/2

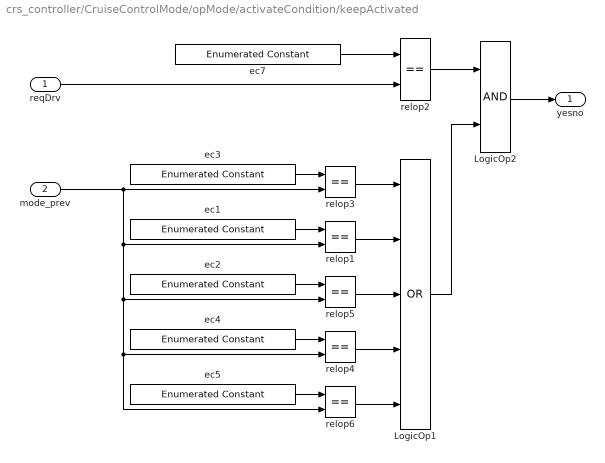
== system crs_controller/CruiseControlMode/opMode/activateCondition/keepActivated ==
  reqDrv : Inport
  mode_prev : Inport  Port=2
  LogicOp1 : Logic  Operator=OR  Inputs=5  AllPortsSameDT=off  OutDataTypeStr=boolean
  LogicOp2 : Logic  AllPortsSameDT=off  OutDataTypeStr=boolean
  ec1 : simulink/Sources/Enumerated Constant  OutDataTypeStr=Enum: opMode  Value=opMode.Increment  SampleTime=inf
  ec2 : simulink/Sources/Enumerated Constant  OutDataTypeStr=Enum: opMode  Value=opMode.IncrementHold  SampleTime=inf
  ec3 : simulink/Sources/Enumerated Constant  OutDataTypeStr=Enum: opMode  Value=opMode.Activate  SampleTime=inf
  ec4 : simulink/Sources/Enumerated Constant  OutDataTypeStr=Enum: opMode  Value=opMode.Decrement  SampleTime=inf
  ec5 : simulink/Sources/Enumerated Constant  OutDataTypeStr=Enum: opMode  Value=opMode.DecrementHold  SampleTime=inf
  ec7 : simulink/Sources/Enumerated Constant  OutDataTypeStr=Enum: reqMode  Value=reqMode.NoRequest  SampleTime=inf
  relop{1..6} (6 alike) : RelationalOperator  Operator===  OutDataTypeStr=boolean  InputSameDT=off
  yesno : Outport  VectorParamsAs1DForOutWhenUnconnected=off
  wires:
  LogicOp1/1 -> LogicOp2/2
  relop2/1 -> LogicOp2/1
  relop6/1 -> LogicOp1/5
  ec5/1 -> relop6/1
  mode_prev/1 -> relop3/2, relop1/2, relop5/2, relop4/2, relop6/2
  relop4/1 -> LogicOp1/4
  relop5/1 -> LogicOp1/3
  ec4/1 -> relop4/1
  ec2/1 -> relop5/1
  ec7/1 -> relop2/1
  ec1/1 -> relop1/1
  ec3/1 -> relop3/1
  relop1/1 -> LogicOp1/2
  relop3/1 -> LogicOp1/1
  reqDrv/1 -> relop2/2
  LogicOp2/1 -> yesno/1

== system crs_controller/CruiseControlMode/opMode/activateCondition/resumeToActive ==
  mode_prev : Inport
  ec3 : simulink/Sources/Enumerated Constant  OutDataTypeStr=Enum: opMode  Value=opMode.Resume  SampleTime=inf
  relop2 : RelationalOperator  Operator===  OutDataTypeStr=boolean  InputSameDT=off
  yesno : Outport  VectorParamsAs1DForOutWhenUnconnected=off
  wires:
  mode_prev/1 -> relop2/2
  ec3/1 -> relop2/1
  relop2/1 -> yesno/1

== system crs_controller/CruiseControlMode/opMode/activateCondition/waitingForButtonHolding ==
  reqDrv : Inport
  LogicOp6 : Logic  Operator=OR  AllPortsSameDT=off  OutDataTypeStr=boolean
  ec10 : Subsystem  DialogController=Simulink.DDGSource  mask(Enumerated Constant){OutDataTypeStr=Enum: reqMode, Value=reqMode.Dec_Middle, SampleTime=inf}
      mask prompts: OutDataTypeStr "Simulink:blkprm_prompts:OutputDataType"; Value "Simulink:blkprm_prompts:ConstConstValue"; SampleTime "Simulink:blkprm_prompts:AllSrcBlksSampleTime"
      mask init:
      | % NOTE:
      | % Value parameter is not evaluated to avoid caching an instance
      | % of the enumeration class by the mask infrastructure.
      | 
      | % Get expression for OutDataTypeStr before evaluation
      | OutDataTypeStr = get_param(gcbh, 'OutDataTypeStr');
      | 
      | % Check data type & value
      | enumconst_cb('MaskInit', OutDataTypeStr, slResolve(Value, gcb));
      | 
      | % Set mask parameter values directly on underlying block
      | % and clear mask workspace variables to prevent underlying
      | % blocks from resolving to unevaluated mask variables.
      | set_param([gcb, '/Constant'], ...
      |     'OutDataTypeStr', OutDataTypeStr, ...
      |     'SampleTime',     SampleTime, ...
      |     'Value',          Value);
      | clear OutDataTypeStr SampleTime Value;
      mask Display:
      | % Get string to use for display purposes
      | enumConstDispStr = get_param(gcbh, 'Value');
      | if isempty(enumConstDispStr)
      | 
      | 				    end
      | disp(enumConstDispStr)
  ec8 : Subsystem  DialogController=Simulink.DDGSource  mask(Enumerated Constant){OutDataTypeStr=Enum: reqMode, Value=reqMode.Inc_Middle, SampleTime=inf}
      mask prompts: OutDataTypeStr "Simulink:blkprm_prompts:OutputDataType"; Value "Simulink:blkprm_prompts:ConstConstValue"; SampleTime "Simulink:blkprm_prompts:AllSrcBlksSampleTime"
      mask init: same as crs_controller/CruiseControlMode/opMode/activateCondition/waitingForButtonHolding/ec10
      mask Display:
      | % Get string to use for display purposes
      | enumConstDispStr = get_param(gcbh, 'Value');
      | if isempty(enumConstDispStr)
      | 
      | 				    end
      | disp(enumConstDispStr)
  relop10 : RelationalOperator  Operator===  OutDataTypeStr=boolean  InputSameDT=off
  relop11 : RelationalOperator  Operator===  OutDataTypeStr=boolean  InputSameDT=off
  yesno : Outport  VectorParamsAs1DForOutWhenUnconnected=off
  wires:
  ec8/1(Out) -> relop10/1
  relop10/1 -> LogicOp6/1
  ec10/1(Out) -> relop11/1
  relop11/1 -> LogicOp6/2
  reqDrv/1 -> relop10/2, relop11/2
  LogicOp6/1 -> yesno/1

== system crs_controller/CruiseControlMode/opMode/disableCondition/buttonsShouldBeCalledWhenActivated ==
  ccsw_request : Inport
  mode_prev : Inport  Port=2
  LogicOp1 : Logic  AllPortsSameDT=off  OutDataTypeStr=boolean
  LogicOp2 : Logic  AllPortsSameDT=off  OutDataTypeStr=boolean
  ec1 : simulink/Sources/Enumerated Constant  OutDataTypeStr=Enum: reqMode  Value=reqMode.Cruise  SampleTime=inf
  ec2 : simulink/Sources/Enumerated Constant  OutDataTypeStr=Enum: reqMode  Value=reqMode.Set  SampleTime=inf
  ec9 : simulink/Sources/Enumerated Constant  OutDataTypeStr=Enum: opMode  Value=opMode.Disable  SampleTime=inf
  relop1 : RelationalOperator  Operator=~=  OutDataTypeStr=boolean  InputSameDT=off
  relop7 : RelationalOperator  Operator===  OutDataTypeStr=boolean  InputSameDT=off
  relop8 : RelationalOperator  Operator=~=  OutDataTypeStr=boolean  InputSameDT=off
  yesno : Outport  VectorParamsAs1DForOutWhenUnconnected=off
  wires:
  ec9/1 -> relop7/1
  ec1/1 -> relop8/1
  relop8/1 -> LogicOp1/1
  LogicOp1/1 -> LogicOp2/1
  relop7/1 -> LogicOp2/2
  LogicOp2/1 -> yesno/1
  mode_prev/1 -> relop7/2
  ccsw_request/1 -> relop1/2, relop8/2
  relop1/1 -> LogicOp1/2
  ec2/1 -> relop1/1

== system crs_controller/CruiseControlMode/opMode/disableCondition/turnOffCruise ==
  ccsw_request : Inport
  mode_prev : Inport  Port=2
  LogicOp2 : Logic  AllPortsSameDT=off  OutDataTypeStr=boolean
  ec1 : simulink/Sources/Enumerated Constant  OutDataTypeStr=Enum: reqMode  Value=reqMode.Cruise  SampleTime=inf
  ec9 : simulink/Sources/Enumerated Constant  OutDataTypeStr=Enum: opMode  Value=opMode.Disable  SampleTime=inf
  relop7 : RelationalOperator  Operator=~=  OutDataTypeStr=boolean  InputSameDT=off
  relop8 : RelationalOperator  Operator===  OutDataTypeStr=boolean  InputSameDT=off
  yesno : Outport  VectorParamsAs1DForOutWhenUnconnected=off
  wires:
  ccsw_request/1 -> relop8/2
  mode_prev/1 -> relop7/2
  LogicOp2/1 -> yesno/1
  relop7/1 -> LogicOp2/2
  relop8/1 -> LogicOp2/1
  ec1/1 -> relop8/1
  ec9/1 -> relop7/1

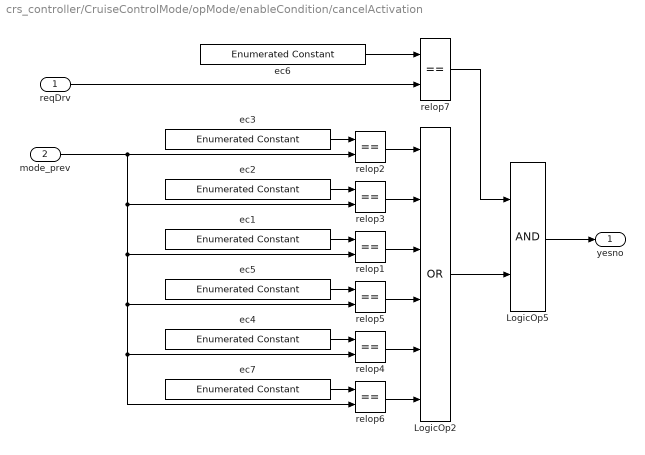
== system crs_controller/CruiseControlMode/opMode/enableCondition/cancelActivation ==
  reqDrv : Inport
  mode_prev : Inport  Port=2
  LogicOp2 : Logic  Operator=OR  Inputs=6  AllPortsSameDT=off  OutDataTypeStr=boolean
  LogicOp5 : Logic  AllPortsSameDT=off  OutDataTypeStr=boolean
  ec1 : simulink/Sources/Enumerated Constant  OutDataTypeStr=Enum: opMode  Value=opMode.IncrementHold  SampleTime=inf
  ec2 : simulink/Sources/Enumerated Constant  OutDataTypeStr=Enum: opMode  Value=opMode.Increment  SampleTime=inf
  ec3 : simulink/Sources/Enumerated Constant  OutDataTypeStr=Enum: opMode  Value=opMode.Activate  SampleTime=inf
  ec4 : simulink/Sources/Enumerated Constant  OutDataTypeStr=Enum: opMode  Value=opMode.DecrementHold  SampleTime=inf
  ec5 : simulink/Sources/Enumerated Constant  OutDataTypeStr=Enum: opMode  Value=opMode.Decrement  SampleTime=inf
  ec6 : simulink/Sources/Enumerated Constant  OutDataTypeStr=Enum: reqMode  Value=reqMode.Cancel  SampleTime=inf
  ec7 : simulink/Sources/Enumerated Constant  OutDataTypeStr=Enum: opMode  Value=opMode.Resume  SampleTime=inf
  relop{1..7} (7 alike) : RelationalOperator  Operator===  OutDataTypeStr=boolean  InputSameDT=off
  yesno : Outport  VectorParamsAs1DForOutWhenUnconnected=off
  wires:
  ec6/1 -> relop7/1
  relop1/1 -> LogicOp2/3
  relop2/1 -> LogicOp2/1
  relop3/1 -> LogicOp2/2
  relop4/1 -> LogicOp2/5
  relop5/1 -> LogicOp2/4
  ec1/1 -> relop1/1
  ec5/1 -> relop5/1
  ec4/1 -> relop4/1
  ec2/1 -> relop3/1
  ec3/1 -> relop2/1
  LogicOp5/1 -> yesno/1
  reqDrv/1 -> relop7/2
  mode_prev/1 -> relop3/2, relop1/2, relop5/2, relop6/2, relop4/2, relop2/2
  LogicOp2/1 -> LogicOp5/2
  relop7/1 -> LogicOp5/1
  ec7/1 -> relop6/1
  relop6/1 -> LogicOp2/6

== system crs_controller/CruiseControlMode/opMode/enableCondition/pressSetSw ==
  reqDrv : Inport
  ec8 : simulink/Sources/Enumerated Constant  OutDataTypeStr=Enum: reqMode  Value=reqMode.Cruise  SampleTime=inf
  relop6 : RelationalOperator  Operator===  OutDataTypeStr=boolean  InputSameDT=off
  yesno : Outport  VectorParamsAs1DForOutWhenUnconnected=off
  wires:
  ec8/1 -> relop6/1
  reqDrv/1 -> relop6/2
  relop6/1 -> yesno/1

== system crs_controller/CruiseControlMode/opMode/resumeCondition/enableToResume ==
  reqDrv : Inport
  mode_prev : Inport  Port=2
  LogicOp1 : Logic  AllPortsSameDT=off  OutDataTypeStr=boolean
  ec15 : simulink/Sources/Enumerated Constant  OutDataTypeStr=Enum: reqMode  Value=reqMode.ResumeReq  SampleTime=inf
  ec3 : simulink/Sources/Enumerated Constant  OutDataTypeStr=Enum: opMode  Value=opMode.Enable  SampleTime=inf
  relop1 : RelationalOperator  Operator===  OutDataTypeStr=boolean  InputSameDT=off
  relop11 : RelationalOperator  Operator===  OutDataTypeStr=boolean  InputSameDT=off
  yesno : Outport  VectorParamsAs1DForOutWhenUnconnected=off
  wires:
  ec15/1 -> relop11/1
  reqDrv/1 -> relop11/2
  relop11/1 -> LogicOp1/1
  mode_prev/1 -> relop1/2
  relop1/1 -> LogicOp1/2
  ec3/1 -> relop1/1
  LogicOp1/1 -> yesno/1

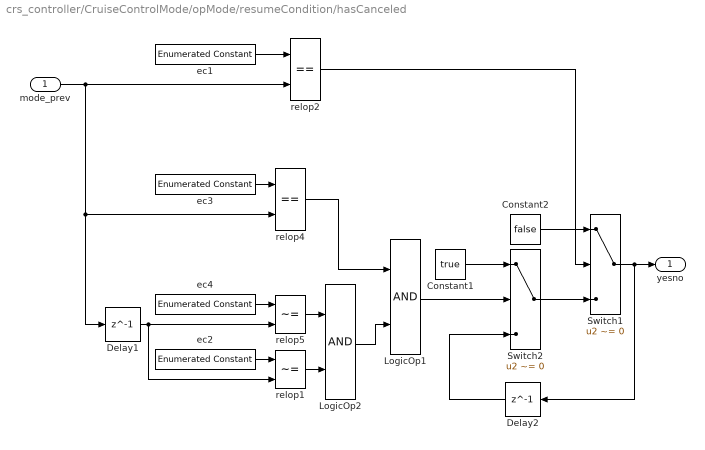
== system crs_controller/CruiseControlMode/opMode/resumeCondition/hasCanceled ==
  mode_prev : Inport
  Constant1 : Constant  Value=true  OutDataTypeStr=boolean
  Constant2 : Constant  Value=false  OutDataTypeStr=boolean
  Delay1 : Delay  DelayLength=1  InitialCondition=opMode.Disable
      settings: AttributesFormatString=Init=%<InitialCondition>
  Delay2 : Delay  DelayLength=1  InitialCondition=false
      settings: AttributesFormatString=Init=%<InitialCondition>
  LogicOp1 : Logic  AllPortsSameDT=off  OutDataTypeStr=boolean
  LogicOp2 : Logic  AllPortsSameDT=off  OutDataTypeStr=boolean
  Switch1 : Switch  Criteria=u2 ~= 0  SaturateOnIntegerOverflow=off  InputSameDT=off
  Switch2 : Switch  Criteria=u2 ~= 0  SaturateOnIntegerOverflow=off  InputSameDT=off
  ec1 : simulink/Sources/Enumerated Constant  OutDataTypeStr=Enum: opMode  Value=opMode.Disable  SampleTime=inf
  ec2 : simulink/Sources/Enumerated Constant  OutDataTypeStr=Enum: opMode  Value=opMode.Enable  SampleTime=inf
  ec3 : simulink/Sources/Enumerated Constant  OutDataTypeStr=Enum: opMode  Value=opMode.Enable  SampleTime=inf
  ec4 : simulink/Sources/Enumerated Constant  OutDataTypeStr=Enum: opMode  Value=opMode.Disable  SampleTime=inf
  relop1 : RelationalOperator  Operator=~=  OutDataTypeStr=boolean  InputSameDT=off
  relop2 : RelationalOperator  Operator===  OutDataTypeStr=boolean  InputSameDT=off
  relop4 : RelationalOperator  Operator===  OutDataTypeStr=boolean  InputSameDT=off
  relop5 : RelationalOperator  Operator=~=  OutDataTypeStr=boolean  InputSameDT=off
  yesno : Outport  VectorParamsAs1DForOutWhenUnconnected=off
  wires:
  ec3/1 -> relop4/1
  ec4/1 -> relop5/1
  LogicOp1/1 -> Switch2/2
  Delay2/1 -> Switch2/3
  Constant1/1 -> Switch2/1
  relop4/1 -> LogicOp1/1
  Switch1/1 -> yesno/1, Delay2/1
  Constant2/1 -> Switch1/1
  Switch2/1 -> Switch1/3
  relop2/1 -> Switch1/2
  ec1/1 -> relop2/1
  mode_prev/1 -> relop2/2, Delay1/1, relop4/2
  ec2/1 -> relop1/1
  relop5/1 -> LogicOp2/1
  relop1/1 -> LogicOp2/2
  LogicOp2/1 -> LogicOp1/2
  Delay1/1 -> relop1/2, relop5/2

== system crs_controller/TargetSpeedThrottle/activated/getThrottleValue/PI controller ==
  targetSpIn : Inport
  vehSp : Inport  Port=2
  Enable : EnablePort  StatesWhenEnabling=reset
  Add : Sum  Inputs=+-
  "DTI " : DiscreteIntegrator  gainval=Ki  SampleTime=Ts  ICPrevOutput=DiscIntNeverNeededParam  ICPrevScaledInput=DiscIntNeverNeededParam
  Kp : Gain  Gain=Kp
  Sum : Sum  Inputs=|++
  throt : Outport  OutputWhenDisabled=reset  InitialOutput=0  VectorParamsAs1DForOutWhenUnconnected=off
  wires:
  Kp/1 -> Sum/1
  "DTI "/1 -> Sum/2
  Sum/1 -> throt/1
  Add/1 -> "DTI "/1, Kp/1
  targetSpIn/1 -> Add/1
  vehSp/1 -> Add/2

== system crs_controller/TargetSpeedThrottle/activated/getThrottleValue/UsePI ==
  throtPI : Inport
  targetSpIn : Inport  Port=2
  vehSp : Inport  Port=3
  throtDrv : Inport  Port=4
  Logical Operator : Logic  AllPortsSameDT=off  OutDataTypeStr=boolean
  Relational Operator : RelationalOperator  OutDataTypeStr=boolean  InputSameDT=off
  relop : RelationalOperator  Operator=>  OutDataTypeStr=boolean  InputSameDT=off
  yesno : Outport  VectorParamsAs1DForOutWhenUnconnected=off
  wires:
  Relational Operator/1 -> Logical Operator/1
  relop/1 -> Logical Operator/2
  Logical Operator/1 -> yesno/1
  throtDrv/1 -> Relational Operator/2
  targetSpIn/1 -> relop/1
  vehSp/1 -> relop/2
  throtPI/1 -> Relational Operator/1

== system crs_controller/CruiseControlMode/opMode/activateCondition/waitingForButtonHolding/ec10 ==
  Constant : Constant  DialogController=Simulink.DDGSource  Value=reqMode.Dec_Middle  OutDataTypeStr=Enum: reqMode  LockScale=on
  Out : Outport  VectorParamsAs1DForOutWhenUnconnected=off
  wires:
  Constant/1 -> Out/1

== system crs_controller/CruiseControlMode/opMode/activateCondition/waitingForButtonHolding/ec8 ==
  Constant : Constant  DialogController=Simulink.DDGSource  Value=reqMode.Inc_Middle  OutDataTypeStr=Enum: reqMode  LockScale=on
  Out : Outport  VectorParamsAs1DForOutWhenUnconnected=off
  wires:
  Constant/1 -> Out/1

== matlab function crs_controller/DriverSwRequest/increment/counter/counter ==
  data: in input boolean size=1; out output boolean size=1; CountValue input uint8 size=1
function out = counter(in,CountValue)
%#codegen

persistent cnt;

% initialize
if isempty(cnt)
    cnt = cast(0,'like',CountValue);
end

% if enabled
if in
    % Output true if CountValue is reached
    if cnt >= CountValue
        out = true;
    else
        % Continue counting up and output false
        cnt = cnt + cast(1,'like',CountValue);
        out = false;
    end
else
    % if disabled, output false and reset
    cnt = cast(0,'like',CountValue);
    out = false;
end

== matlab function crs_controller/DriverSwRequest/decrement/counter/counter ==
  data: in input boolean size=1; out output boolean size=1; CountValue input uint8 size=1
function out = counter(in,CountValue)
%#codegen

persistent cnt;

% initialize
if isempty(cnt)
    cnt = cast(0,'like',CountValue);
end

% if enabled
if in
    % Output true if CountValue is reached
    if cnt >= CountValue
        out = true;
    else
        % Continue counting and output false        
        cnt = cnt + cast(1,'like',CountValue);
        out = false;
    end
else
    % if disabled, output false and reset
    cnt = cast(0,'like',CountValue);
    out = false;
end
